simulink model "DABTestHarnessPlant"  (R2026a)
settings: Solver=ode23t  StopTime=5e-3  MaxStep=1e-5  AbsTol=1e-3
PreLoadFcn:
  | DABDefaultInputParameters;
model workspace (MAT data in the model file):
  ConverterKey = "DAB"
undefined symbols (not defined in the file or in its folder): DABController, DABDesign, DiscIntNeverNeededParam
libraries: ee_lib x45, nesl_utility x38, fl_lib x19, simulink_extras x1
(part 1 of 4)
settings Model: Creator=vsolaise  LastModifiedBy=vsolaise
settings SimscapeCC: SimscapeNominalValues="[{\"value\":\"1\",\"unit\":\"A\"},{\"value\":\"1\",\"unit\":\"bar\"},{\"value\":\"1\",\"unit\":\"cm^2\"},{\"value\":\"1\",\"unit\":\"cm^3/s\"},{\"value\":\"1\",\"unit\":\"kJ/kg\"},{\"value\":\"1\",\"unit\":\"kW\"},{\"value\":\"1\",\"unit\":\"l\"},{\"value\":\"1\",\"unit\":\"N\"},{\"value\":\"1\",\"unit\":\"N*m\"},{\"value\":\"1\",\"unit\":\"V\"}]"  SimscapeLogName=simlogDABConverter  SimscapeLogDataHistory=5000.0

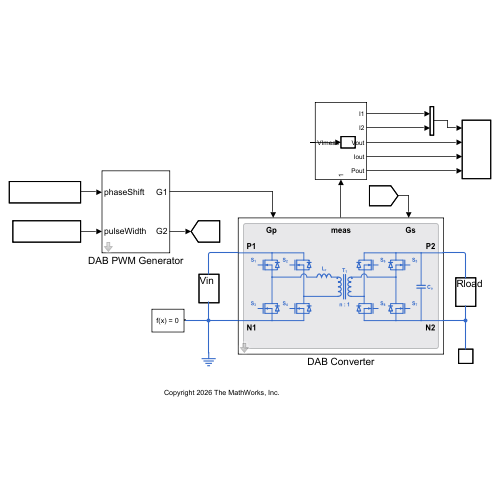
[thumbnail: Simulink's stored preview of the top-level diagram]
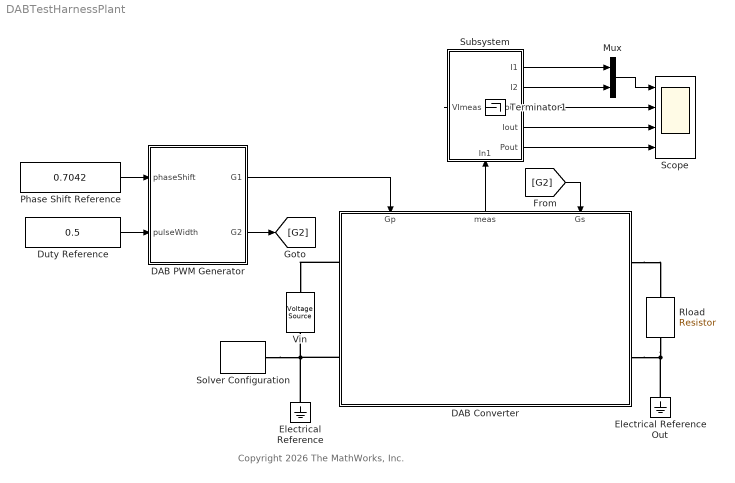
== system DABTestHarnessPlant ==
  note: Copyright 2026 The MathWorks, Inc.
  DAB Converter : Subsystem  mask(Dual Active Bridge DC-DC Converter){modelOption=Simplified, ratedPower=10000, ratedPower_unit=W, Vin=750, Vin_unit=V, Vout=525, Vout_unit=V, Fsw=100000, Fsw_unit=Hz, turnsRatio=1.4286, Co=2.963e-5, Co_unit=F, Rco=0.001, Rco_unit=mOhm, seriesInductorOption=Use transformer leakage inductance, Lr=0, Lr_unit=H, RLr=0.01, RLr_unit=Ohm, Lm=1.4062e-3, Lm_unit=H, Llk1=3.913e-5, Llk1_unit=H, RLlk1=0.01, RLlk1_unit=Ohm, Llk2=4.7935e-6, Llk2_unit=H, RLlk2=0.01, RLlk2_unit=Ohm, Vco=525, Vco_unit=V, switchDeviceOptionPri=MOSFET (Ideal, Switching) with Thermal, RdsOnPri=0.005, RdsOnPri_unit=Ohm, GdsOffPri=1e-5, GdsOffPri_unit=1/Ohm, VthPri=3, VthPri_unit=V, CossPri=2e-10, CossPri_unit=F, simTempPri=25, simTempPri_unit=degC, VfPri=0.005, VfPri_unit=V, RdPri=1, RdPri_unit=mOhm, GdPri=1e-5, GdPri_unit=1/Ohm, switchDeviceOptionSec=MOSFET (Ideal, Switching) with Thermal, RdsOnSec=0.005, RdsOnSec_unit=Ohm, GdsOffSec=1e-5, GdsOffSec_unit=1/Ohm, VthSec=3, VthSec_unit=V, CossSec=2e-10, CossSec_unit=F, simTempSec=25, simTempSec_unit=degC, VfSec=0.005, VfSec_unit=V, RdSec=1, RdSec_unit=mOhm, GdSec=1e-5, GdSec_unit=1/Ohm}
      mask prompts: modelOption "Model option"; ratedPower "Rated power"; Vin "Nominal input voltage"; Vout "Nominal output voltage"; Fsw "Switching frequency"; turnsRatio "Transformer turns ratio (Np/Ns)"; Co "Secondary output capacitance"; Rco "Secondary output capacitance ESR"; seriesInductorOption "Series inductance"; Lr "Series inductance (Lr)"; RLr "Series inductance resistance"; Lm "Magnetizing inductance (Lm)"; Llk1 "Primary leakage inductance (Llk1)"; RLlk1 "Primary winding resistance"; Llk2 "Secondary leakage inductance (Llk2)"; RLlk2 "Secondary winding resistance"; Vco "Initial output capacitor voltage"; switchDeviceOptionPri "Switch device"; RdsOnPri "On-state resistance (RdsOn)"; GdsOffPri "Off-state conductance (GdsOff)"; VthPri "Threshold voltage"; CossPri "Output capacitance (Coss)"; simTempPri "Simulation temperature"; VfPri "Diode forward voltage (Vf)"; RdPri "Diode on resistance (Rd)"; GdPri "Diode off conductance (Gd)"; switchDeviceOptionSec "Switch device"; RdsOnSec "On-state resistance (RdsOn)"; GdsOffSec "Off-state conductance (GdsOff)"; VthSec "Threshold voltage"; CossSec "Output capacitance (Coss)"; simTempSec "Simulation temperature"; VfSec "Diode forward voltage (Vf)"; RdSec "Diode on resistance (Rd)"; GdSec "Diode off conductance (Gd)"
      mask help: Dual Active Bridge (DAB) DC-DC Converter with variant options for HDL and Simulation models.
      mask init:
      | %% Unit conversion: convert displayed values to base SI units
      | convMap = containers.Map( ...
      |     {'W','kW','MW','V','kV','mV','F','mF','uF','nF','pF', ...
      |      'H','mH','uH','nH','Ohm','kOhm','mOhm','S','mS','1/Ohm', ...
      |      'Hz','kHz','MHz'}, ...
      |     {1, 1e3, 1e6, 1, 1e3, 1e-3, 1, 1e-3, 1e-6, 1e-9, 1e-12, ...
      |      1, 1e-3, 1e-6, 1e-9, 1, 1e3, 1e-3, 1, 1e-3, 1, ...
      |      1, 1e3, 1e6});
      | 
      | ratedPower_SI = ratedPower * convMap(ratedPower_unit);
      | Vin_SI = Vin * convMap(Vin_unit);
      | Vout_SI = Vout * convMap(Vout_unit);
      | Fsw_SI = Fsw * convMap(Fsw_unit);
      | Llk1_SI = Llk1 * convMap(Llk1_unit);
      | RLlk1_SI = RLlk1 * convMap(RLlk1_unit);
      | Llk2_SI = Llk2 * convMap(Llk2_unit);
      | RLlk2_SI = RLlk2 * convMap(RLlk2_unit);
      | Lr_SI = Lr * convMap(Lr_unit);
      | RLr_SI = RLr * convMap(RLr_unit);
      | % When the model compiles, the transformer leakages must be positive, and so must Lr when the
      | % external inductor is used. A dialog change is not checked, so Lr can be entered after the option.
      | if any(strcmp(get_param(bdroot(gcb), 'SimulationStatus'), {'updating', 'initializing'}))
      |     if ~(isfinite(Llk1_SI) && Llk1_SI > 0 && isfinite(Llk2_SI) && Llk2_SI > 0)
      |         error('The transformer leakage inductances must be positive. Primary: %g H, secondary: %g H.', Llk1_SI, Llk2_SI);
      |     end
      |     if strcmp(get_param(gcb, 'seriesInductorOption'), 'Use external inductance') && ~(isfinite(Lr_SI) && Lr_SI > 0)
      |         error('The external series inductance must be positive when it is used. Lr: %g H.', Lr_SI);
      |     end
      | end
      | Lm_SI = Lm * convMap(Lm_unit);
      | Co_SI = Co * convMap(Co_unit);
      | Rco_SI = Rco * convMap(Rco_unit);
      | Vco_SI = Vco * convMap(Vco_unit);
      | 
      | %% Primary switch params
      | RdsOnPri_SI = RdsOnPri * convMap(RdsOnPri_unit);
      | GdsOffPri_SI = GdsOffPri * convMap(GdsOffPri_unit);
      | VthPri_SI = VthPri * convMap(VthPri_unit);
      | CossPri_SI = CossPri * convMap(CossPri_unit);
      | 
      | %% Secondary switch params
      | RdsOnSec_SI = RdsOnSec * convMap(RdsOnSec_unit);
      | GdsOffSec_SI = GdsOffSec * convMap(GdsOffSec_unit);
      | VthSec_SI = VthSec * convMap(VthSec_unit);
      | CossSec_SI = CossSec * convMap(CossSec_unit);
      | 
      | %% Primary switch protection-diode params
      | VfPri_SI = VfPri * convMap(VfPri_unit);
      | RdPri_SI = RdPri * convMap(RdPri_unit);
      | GdPri_SI = GdPri * convMap(GdPri_unit);
      | 
      | %% Secondary switch protection-diode params
      | VfSec_SI = VfSec * convMap(VfSec_unit);
      | RdSec_SI = RdSec * convMap(RdSec_unit);
      | GdSec_SI = GdSec * convMap(GdSec_unit);
      | 
      | 
      | %% Simulation temperature (thermal MOSFET)
      | % Temperature is an OFFSET unit (K = degC + 273.15), so it cannot use the
      | % multiplicative convMap; convert it explicitly. These Kelvin variables are
      | % read directly by each thermal MOSFET device junction-temperature target and
      | % by each bridge Temperature Source.
      | if strcmp(simTempPri_unit, 'degC')
      |     simTempPri_K = simTempPri + 273.15;
      | else
      |     simTempPri_K = simTempPri;
      | end
      | if strcmp(simTempSec_unit, 'degC')
      |     simTempSec_K = simTempSec + 273.15;
      | else
      |     simTempSec_K = simTempSec;
      | end
      | 
      | %% Apply variant selection
      | selectDABConverterModelOption(gcb);
      settings: CopyFcn="set_param(gcbh,\"LinkStatus\",\"none\");"  PortSchema="{\"entries\":[{\"content\":{\"sides\":[{\"content\":{\"connectorIds\":[\"LConn1\",\"LConn2\"]},\"type\":\"ConnectorPlacement.EquallySpacedRectSide\",\"uuid\":\"5eb81d01-b33d-480d-b92b-9ee197a9667d\"},{\"content\":{\"connectorIds\":[\"RConn1\",\"RConn2\"],\"side\":\"RIGHT\"},\"type\":\"ConnectorPlacement.EquallySpacedRectSide\",\"uuid\":\"a719554b-e33a-474b-8c80-408706add5ae\"},{\"content\":{\"connectorIds\":[\"In1\",\"Out1\",\"In2\"],\"side\":\"TOP\"},\"type\":\"ConnectorPlacement.EquallySpacedRectSide\",\"uuid\":\"aea510b9-aefe-49d3-b91f-0f6ebd0a6b41\"}]},\"type\":\"ConnectorPlacement.EquallySpacedConnector\",\"uuid\":\"00bcdd44-1110-449b-876a-23d9733cbf45\"}],\"packageUris\":[\"http://schema.mathworks.com/mf0/Connector/R2020b\"],\"version\":\"1.0\"}"
      mask Help: web('DABConverter.html')
      mask TypeOptions modelOption: Simplified | Detailed
      mask Callback modelOption: selectDABConverterModelOption(gcb);
      mask TypeOptions ratedPower_unit: W | kW | MW
      mask TypeOptions Vin_unit: mV | V | kV
      mask TypeOptions Vout_unit: mV | V | kV
      mask TypeOptions Fsw_unit: Hz | kHz | MHz
      mask TypeOptions Co_unit: F | mF | uF | nF | pF
      mask TypeOptions Rco_unit: mOhm | Ohm | kOhm
      mask TypeOptions seriesInductorOption: Use external inductance | Use transformer leakage inductance
      mask Callback seriesInductorOption: selectDABSeriesInductor(gcb);
      mask TypeOptions Lr_unit: H | mH | uH | nH
      mask TypeOptions RLr_unit: mOhm | Ohm | kOhm
      mask TypeOptions Lm_unit: H | mH | uH | nH
      mask TypeOptions Llk1_unit: H | mH | uH | nH
      mask TypeOptions RLlk1_unit: mOhm | Ohm | kOhm
      mask TypeOptions Llk2_unit: H | mH | uH | nH
      mask TypeOptions RLlk2_unit: mOhm | Ohm | kOhm
      mask TypeOptions Vco_unit: V | kV | mV
      mask TypeOptions switchDeviceOptionPri: Ideal Switch | MOSFET (Ideal, Switching) with Thermal
      mask Callback switchDeviceOptionPri: selectDABConverterSwitchDevice(gcb)
      mask TypeOptions RdsOnPri_unit: mOhm | Ohm | kOhm
      mask TypeOptions GdsOffPri_unit: S | mS | 1/Ohm
      mask TypeOptions VthPri_unit: mV | V | kV
      mask TypeOptions CossPri_unit: F | mF | uF | nF | pF
      mask TypeOptions simTempPri_unit: degC | K
      mask TypeOptions VfPri_unit: mV | V | kV
      mask TypeOptions RdPri_unit: mOhm | Ohm | kOhm
      mask TypeOptions GdPri_unit: S | mS | 1/Ohm
      mask TypeOptions switchDeviceOptionSec: Ideal Switch | MOSFET (Ideal, Switching) with Thermal
      mask Callback switchDeviceOptionSec: selectDABConverterSwitchDevice(gcb)
      mask TypeOptions RdsOnSec_unit: mOhm | Ohm | kOhm
      mask TypeOptions GdsOffSec_unit: S | mS | 1/Ohm
      mask TypeOptions VthSec_unit: mV | V | kV
      mask TypeOptions CossSec_unit: F | mF | uF | nF | pF
      mask TypeOptions simTempSec_unit: degC | K
      mask TypeOptions VfSec_unit: mV | V | kV
      mask TypeOptions RdSec_unit: mOhm | Ohm | kOhm
      mask TypeOptions GdSec_unit: S | mS | 1/Ohm
      mask DialogControl DABConverterParameters Prompt: DAB Converter Parameters
      mask DialogControl TransformerParameters Prompt: Transformer
      mask DialogControl PrimarySwitch Prompt: Primary Switch
      mask DialogControl openMOSFETPriMask Prompt: Open MOSFET block mask
      mask DialogControl openMOSFETPriMask Callback: open_system([gcb '/DABConverterVariant/DetailedModel/PrimaryBridge/SwitchingMOSFETwithThermal/MOSFETPriA1'], 'mask')
      mask DialogControl applyMOSFETPriParam Prompt: Apply parameters to all primary MOSFET blocks
      mask DialogControl applyMOSFETPriParam Callback: applyDABConverterMOSFETParameters(gcb, 'primary')
      mask DialogControl SecondarySwitch Prompt: Secondary Switch
      mask DialogControl openMOSFETSecMask Prompt: Open MOSFET block mask
      mask DialogControl openMOSFETSecMask Callback: open_system([gcb '/DABConverterVariant/DetailedModel/SecondaryBridge/SwitchingMOSFETwithThermal/MOSFETSecA1'], 'mask')
      mask DialogControl applyMOSFETSecParam Prompt: Apply parameters to all secondary MOSFET blocks
      mask DialogControl applyMOSFETSecParam Callback: applyDABConverterMOSFETParameters(gcb, 'secondary')
      mask DialogControl ExportPanel Prompt: Export to Unmasked Subsystem
      mask DialogControl ExportInfo Prompt: To customize the converter, export it as an unmasked subsystem with the active variant flattened - a standalone, fully-editable circuit plus a parameter file. Requires the "Variant Manager for Simulink" add-on.
      mask DialogControl exportToModel Prompt: Export
      mask DialogControl exportToModel Callback: exportConverterModelFromMask(gcb);
      mask Display: image('DABConverterIcon.svg');
  DAB PWM Generator : Subsystem  mask(Dual Active Bridge PWM Generator){solverMode=Variable-step (continuous), Ts=1e-8, Fsw=DABDesign.switchingFrequency.value, Tdead=DABDesign.deadTime.value, primaryGateVoltageOn=DABController.gateVoltage, primaryGateVoltageOff=0, secondaryGateVoltageOn=DABController.gateVoltage, secondaryGateVoltageOff=0}
      mask prompts: solverMode "Solver mode"; Ts "Sample time (s)"; Fsw "Switching frequency (Hz)"; Tdead "Dead time (s)"; primaryGateVoltageOn "Primary bridge gate ON voltage (V)"; primaryGateVoltageOff "Primary bridge gate OFF voltage (V)"; secondaryGateVoltageOn "Secondary bridge gate ON voltage (V)"; secondaryGateVoltageOff "Secondary bridge gate OFF voltage (V)"
      mask help:
      | This block generates dual-active-bridge PWM gate signals with a dead time from a commanded phase shift.
      |
      | For a variable-step solver, set Solver mode to Variable-step (continuous). For a fixed-step solver, set Solver mode to Fixed-step (discrete) and set Sample time to a positive value.
      mask init:
      | % Solver mode. Switch every sawtooth ramp in this block between its continuous
      | % and its discrete implementation, and show the sample time only when it is used.
      | pwmGeneratorBlock = gcb;
      | if strcmp(get_param(pwmGeneratorBlock, 'solverMode'), 'Fixed-step (discrete)')
      |     pwmGeneratorRampChoice = 'FixedStep';
      |     pwmGeneratorSampleTimeVisibility = 'on';
      | else
      |     pwmGeneratorRampChoice = 'VariableStep';
      |     pwmGeneratorSampleTimeVisibility = 'off';
      | end
      | 
      | % A block may hold more than one ramp, at any depth, so the ramps are found by the
      | % "Ramp Mode" suffix on their names rather than by one fixed path. The match filter
      | % keeps every variant choice in the search, which is also what silences the
      | % find_system default-variants warning.
      | pwmGeneratorRamps = find_system(pwmGeneratorBlock, ...
      |     'MatchFilter', @Simulink.match.allVariants, 'LookUnderMasks', 'all', ...
      |     'FollowLinks', 'on', 'Regexp', 'on', 'BlockType', 'SubSystem', ...
      |     'Name', 'Ramp Mode$');
      | for pwmGeneratorRampIndex = 1:numel(pwmGeneratorRamps)
      |     set_param(pwmGeneratorRamps{pwmGeneratorRampIndex}, ...
      |         'LabelModeActiveChoice', pwmGeneratorRampChoice);
      | end
      | 
      | % Only the discrete ramp declares a rate, so the sample time is hidden in the
      | % continuous mode. The guard keeps the code silent on a mask still being built.
      | pwmGeneratorMask = Simulink.Mask.get(pwmGeneratorBlock);
      | pwmGeneratorSampleTime = pwmGeneratorMask.getParameter('Ts');
      | if ~isempty(pwmGeneratorSampleTime)
      |     pwmGeneratorSampleTime.Visible = pwmGeneratorSampleTimeVisibility;
      | end
      mask Help: web('DABPWMGenerator.html')
      mask TypeOptions solverMode: Variable-step (continuous) | Fixed-step (discrete)
      mask Callback solverMode:
      | % Solver mode. Switch every sawtooth ramp in this block between its continuous
      | % and its discrete implementation, and show the sample time only when it is used.
      | pwmGeneratorBlock = gcb;
      | if strcmp(get_param(pwmGeneratorBlock, 'solverMode'), 'Fixed-step (discrete)')
      |     pwmGeneratorRampChoice = 'FixedStep';
      |     pwmGeneratorSampleTimeVisibility = 'on';
      | else
      |     pwmGeneratorRampChoice = 'VariableStep';
      |     pwmGeneratorSampleTimeVisibility = 'off';
      | end
      | 
      | % A block may hold more than one ramp, at any depth, so the ramps are found by the
      | % "Ramp Mode" suffix on their names rather than by one fixed path. The match filter
      | % keeps every variant choice in the search, which is also what silences the
      | % find_system default-variants warning.
      | pwmGeneratorRamps = find_system(pwmGeneratorBlock, ...
      |     'MatchFilter', @Simulink.match.allVariants, 'LookUnderMasks', 'all', ...
      |     'FollowLinks', 'on', 'Regexp', 'on', 'BlockType', 'SubSystem', ...
      |     'Name', 'Ramp Mode$');
      | for pwmGeneratorRampIndex = 1:numel(pwmGeneratorRamps)
      |     set_param(pwmGeneratorRamps{pwmGeneratorRampIndex}, ...
      |         'LabelModeActiveChoice', pwmGeneratorRampChoice);
      | end
      | 
      | % Only the discrete ramp declares a rate, so the sample time is hidden in the
      | % continuous mode. The guard keeps the code silent on a mask still being built.
      | pwmGeneratorMask = Simulink.Mask.get(pwmGeneratorBlock);
      | pwmGeneratorSampleTime = pwmGeneratorMask.getParameter('Ts');
      | if ~isempty(pwmGeneratorSampleTime)
      |     pwmGeneratorSampleTime.Visible = pwmGeneratorSampleTimeVisibility;
      | end
      mask DialogControl DescTextVar Prompt:
      | This block generates dual-active-bridge PWM gate signals with a dead time from a commanded phase shift.
      | 
      | For a variable-step solver, set Solver mode to Variable-step (continuous). For a fixed-step solver, set Solver mode to Fixed-step (discrete) and set Sample time to a positive value.
      mask DialogControl SolverPanel Prompt: Solver Settings
      mask DialogControl SwitchingPanel Prompt: Switching Parameters
      mask DialogControl GateDrivePanel Prompt: Gate Drive
  Duty Reference : Constant  Value=0.5
  Electrical Reference : fl_lib/Electrical/Electrical Elements/Electrical Reference
  Electrical Reference Out : fl_lib/Electrical/Electrical Elements/Electrical Reference
  Mux : Mux  Inputs=2
  Phase Shift Reference : Constant  Value=0.7042
  Rload : fl_lib/Electrical/Electrical Elements/Resistor  R=27.5625 Ohm  i_specify=off  i_priority=None  i=0 A  i_nominal_specify=off  i_nominal_value=1  i_nominal_unit=A  v_specify=off  v_priority=None  v=0 V  v_nominal_specify=off  v_nominal_value=1  v_nominal_unit=V
  Scope : Scope  NumInputPorts=4
      settings: Title=Output Voltage (V)  ActiveDisplayYMinimum=384.33567337339571  ActiveDisplayYMaximum=543.59763143317582
  Solver Configuration : nesl_utility/Solver Configuration  PhysicalDomain=network_engine_domain  SubClassName=solver  LeftPortType=input  RightPortType=generic  Tones=[]  Harmonics=[]  SimulateNoise=off  Profile=off  UseLocalSampling=off  EnableSwitchedLinearOptims=on  FrequencyDomain=off  UseCCode=off  RelTol=0.001  AbsTol=0.001  MinStep=1e-09  ToWorkspace=off  RevertToSquareIcSolve=off  NumHomotopyIterations=100  PhasorMode=off  PhasorModeNumHarmonics=1  ConsistencySolver=NEWTON_XTOL_AFTER_FTOL  CanonicalOrdering=UNORDERED  OptimizeIntermediates=UNOPTIMIZED  IndexReductionMethod=DerivativeReplacement  DoDC=off  ResidualTolerance=1e-09  ConsistencyTolSource=GLOBAL  ConsistencyAbsTol=0.001  ConsistencyRelTol=0.001  ConsistencyTolFactor=0.001  UseLocalSolver=on  LocalSolverChoice=NE_BACKWARD_EULER_ADVANCER  ResolveIndetEquations=on  FunctionEvalNumThread=1  LocalSolverSampleTime=1e-7  DoFixedCost=on  MaxNonlinIter=6  MaxModeIter=2  ComputeImpulses=off  ImpulseIterations=2  LinearAlgebra=auto  LinearAlgebraNumThread=0  EquationFormulation=NE_TIME_EF  DelaysMemoryBudget=1024  AutomaticFiltering=on  FilteringTimeConstant=0.001  PartitionStorageMethod=AS_NEEDED  PartitionMemoryBudget=1024  PartitionMethod=ROBUST  MultibodyUseLocalSolver=off  MultibodyLocalSolverChoice=ODE1  MultibodyLocalSolverSampleTime=0.001
  Subsystem : Subsystem
      settings: PortSchema="{\"entries\":[{\"content\":{\"sides\":[{\"content\":{\"connectorIds\":[\"Out6\"]},\"type\":\"ConnectorPlacement.EquallySpacedRectSide\",\"uuid\":\"f2b899f7-a6f0-4063-b280-75fc43e532d5\"},{\"content\":{\"connectorIds\":[\"Out1\",\"Out2\",\"Out3\",\"Out4\",\"Out5\"],\"side\":\"RIGHT\"},\"type\":\"ConnectorPlacement.EquallySpacedRectSide\",\"uuid\":\"5de70531-a79e-4c62-9cd6-16ab34a78e6e\"},{\"content\":{\"side\":\"TOP\"},\"type\":\"ConnectorPlacement.EquallySpacedRectSide\",\"uuid\":\"e5bc4a57-59c4-404a-a3d7-aeb4f7590bd8\"},{\"content\":{\"connectorIds\":[\"In1\"],\"side\":\"BOTTOM\"},\"type\":\"ConnectorPlacement.EquallySpacedRectSide\",\"uuid\":\"d1dcebc2-7af2-4d54-9158-2e062e509fbc\"}]},\"type\":\"ConnectorPlacement.EquallySpacedConnector\",\"uuid\":\"ad567749-1bde-47d1-aaf1-1f8d8a2cad80\"}],\"packageUris\":[\"http://schema.mathworks.com/mf0/Connector/R2020b\"],\"version\":\"1.0\"}"
  Terminator1 : Terminator
  Vin : ee_lib/Sources/Voltage Source  dc_voltage=750 V  ac_voltage=0 V  ac_shift=0 rad  ac_frequency=60 Hz  noise_mode=ee.enum.sources.noise.Disabled  PSD=0 V^2/Hz  sample_time=1e-3 s  repeatability=ee.enum.sources.repeatability.NotRepeatable  user_seed=0  auto_seed=1556750757  i_specify=off  i_priority=None  i=0 A  i_nominal_specify=off  i_nominal_value=1  i_nominal_unit=A  v_specify=off  v_priority=None  v=0 V  v_nominal_specify=off  v_nominal_value=1  v_nominal_unit=V
  wires:
  Subsystem/1(I1) -> Mux/1
  Subsystem/2(I2) -> Mux/2
  DAB Converter/1(meas) -> Subsystem/1(In1)
  Subsystem/3(Vout) -> Scope/2
  Mux/1 -> Scope/1
  Subsystem/4(Iout) -> Scope/3
  Subsystem/5(Pout) -> Scope/4
  Phase Shift Reference/1 -> DAB PWM Generator/1(phaseShift)
  Duty Reference/1 -> DAB PWM Generator/2(pulseWidth)
  DAB PWM Generator/1(G1) -> DAB Converter/1(Gp)
  Subsystem/6(VImeas) -> Terminator1/1
  DAB PWM Generator/2(G2) -> [G2]
  [G2] -> DAB Converter/2(Gs)
  connections:
  DAB Converter/LConn1 -- Vin/LConn1
  DAB Converter/RConn1 -- Rload/LConn1
  Solver Configuration/RConn1 -- Electrical Reference/LConn1 -- DAB Converter/LConn2 -- Vin/RConn1
  Rload/RConn1 -- Electrical Reference Out/LConn1 -- DAB Converter/RConn2

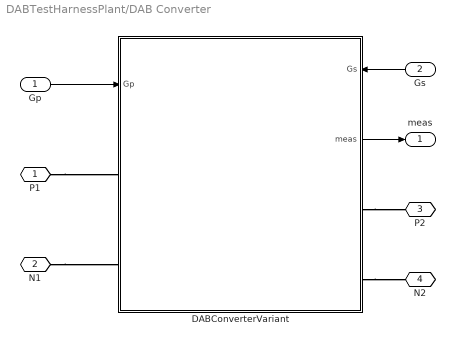
== system DABTestHarnessPlant/DAB Converter ==
  Gp : Inport
  Gs : Inport  Port=2
  DABConverterVariant : Subsystem  Variant=on  VariantControlMode=label  LabelModeActiveChoice=SimplifiedModel
      settings: PortSchema="{\"entries\":[{\"content\":{\"sides\":[{\"content\":{\"connectorIds\":[\"In1\",\"LConn1\",\"LConn2\"]},\"type\":\"ConnectorPlacement.EquallySpacedRectSide\",\"uuid\":\"6f245ee7-ecea-433e-8ace-55b7238b8bbd\"},{\"content\":{\"connectorIds\":[\"In2\",\"Out1\",\"RConn1\",\"RConn2\"],\"side\":\"RIGHT\"},\"type\":\"ConnectorPlacement.EquallySpacedRectSide\",\"uuid\":\"af7f8c88-8cd1-4285-8228-b98ea57f06ae\"},{\"content\":{\"side\":\"TOP\"},\"type\":\"ConnectorPlacement.EquallySpacedRectSide\",\"uuid\":\"820d378e-11b2-4797-9989-1ab18f65f7f5\"}]},\"type\":\"ConnectorPlacement.EquallySpacedConnector\",\"uuid\":\"ae0f71da-cdc3-4120-89e7-21ff59b441bf\"}],\"packageUris\":[\"http://schema.mathworks.com/mf0/Connector/R2020b\"],\"version\":\"1.0\"}"
  P1 : PMIOPort  Side=Left
  N1 : PMIOPort  Port=2  Side=Left
  P2 : PMIOPort  Port=3  Side=Right
  N2 : PMIOPort  Port=4  Side=Right
  meas : Outport
  wires:
  Gp/1 -> DABConverterVariant/1(Gp)
  Gs/1 -> DABConverterVariant/2(Gs)
  DABConverterVariant/1(meas) -> meas/1
  connections:
  DABConverterVariant/RConn2 -- N2/RConn1
  DABConverterVariant/RConn1 -- P2/RConn1
  N1/RConn1 -- DABConverterVariant/LConn2
  P1/RConn1 -- DABConverterVariant/LConn1

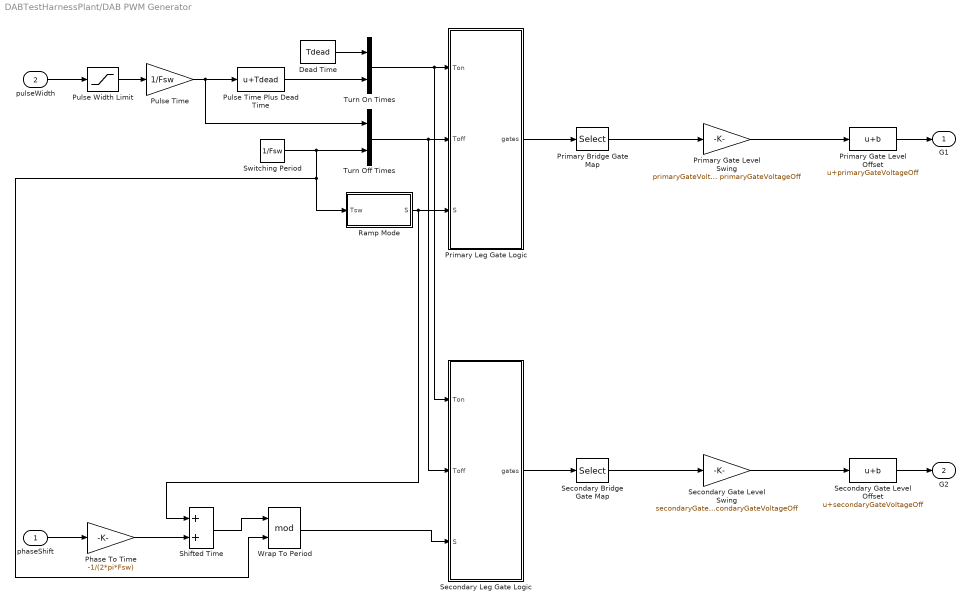
== system DABTestHarnessPlant/DAB PWM Generator ==
  phaseShift : Inport
  pulseWidth : Inport  Port=2
  Dead Time : Constant  Value=Tdead
  Phase To Time : Gain  Gain=-1/(2*pi*Fsw)
  Primary Bridge Gate Map : Selector  InputPortWidth=2  IndexOptions=Index vector (dialog)  Indices=[1 2 2 1]  OutputSizes=1
  Primary Gate Level Offset : Bias  Bias=primaryGateVoltageOff
  Primary Gate Level Swing : Gain  Gain=primaryGateVoltageOn - primaryGateVoltageOff
  Primary Leg Gate Logic : Subsystem
  Pulse Time : Gain  Gain=1/Fsw
  Pulse Time Plus Dead Time : Bias  Bias=Tdead
  Pulse Width Limit : Saturate  UpperLimit=1 - Tdead*Fsw  LowerLimit=Tdead*Fsw
  Ramp Mode : Subsystem  Variant=on  VariantControlMode=label  LabelModeActiveChoice=VariableStep
  Secondary Bridge Gate Map : Selector  InputPortWidth=2  IndexOptions=Index vector (dialog)  Indices=[1 2 2 1]  OutputSizes=1
  Secondary Gate Level Offset : Bias  Bias=secondaryGateVoltageOff
  Secondary Gate Level Swing : Gain  Gain=secondaryGateVoltageOn - secondaryGateVoltageOff
  Secondary Leg Gate Logic : Subsystem
  Shifted Time : Sum
  Switching Period : Constant  Value=1/Fsw
  Turn Off Times : Mux  Inputs=2
  Turn On Times : Mux  Inputs=2
  Wrap To Period : Math  Operator=mod
  G1 : Outport
  G2 : Outport  Port=2
  wires:
  Secondary Gate Level Offset/1 -> G2/1
  Primary Gate Level Offset/1 -> G1/1
  Secondary Bridge Gate Map/1 -> Secondary Gate Level Swing/1
  Secondary Leg Gate Logic/1(gates) -> Secondary Bridge Gate Map/1
  Primary Bridge Gate Map/1 -> Primary Gate Level Swing/1
  Primary Leg Gate Logic/1(gates) -> Primary Bridge Gate Map/1
  Wrap To Period/1 -> Secondary Leg Gate Logic/3(S)
  Shifted Time/1 -> Wrap To Period/1
  Phase To Time/1 -> Shifted Time/2
  phaseShift/1 -> Phase To Time/1
  Ramp Mode/1(S) -> Shifted Time/1, Primary Leg Gate Logic/3(S)
  Turn Off Times/1 -> Secondary Leg Gate Logic/2(Toff), Primary Leg Gate Logic/2(Toff)
  Turn On Times/1 -> Secondary Leg Gate Logic/1(Ton), Primary Leg Gate Logic/1(Ton)
  Secondary Gate Level Swing/1 -> Secondary Gate Level Offset/1
  Primary Gate Level Swing/1 -> Primary Gate Level Offset/1
  Switching Period/1 -> Wrap To Period/2, Ramp Mode/1(Tsw), Turn Off Times/2
  Pulse Time Plus Dead Time/1 -> Turn On Times/2
  Dead Time/1 -> Turn On Times/1
  Pulse Time/1 -> Turn Off Times/1, Pulse Time Plus Dead Time/1
  Pulse Width Limit/1 -> Pulse Time/1
  pulseWidth/1 -> Pulse Width Limit/1

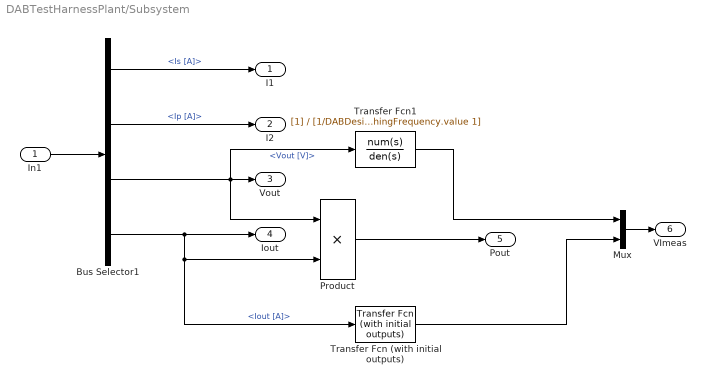
== system DABTestHarnessPlant/Subsystem ==
  In1 : Inport
  Bus Selector1 : BusSelector  OutputSignals=Is [A],Ip [A],Vout [V],Iout [A]
  Mux : Mux  Inputs=2
  Product : Product
  Transfer Fcn (with initial outputs) : simulink_extras/Additional Linear/Transfer Fcn (with initial outputs)  N=[1]  D=[1/DABDesign.switchingFrequency.value 1]  Y0=DABDesign.V2nom.value  U0=DABDesign.V2nom.value
  Transfer Fcn1 : TransferFcn  Denominator=[1/DABDesign.switchingFrequency.value 1]
  I1 : Outport
  I2 : Outport  Port=2
  Vout : Outport  Port=3
  Iout : Outport  Port=4
  Pout : Outport  Port=5
  VImeas : Outport  Port=6
  wires:
  In1/1 -> Bus Selector1/1
  Bus Selector1/1 -> I1/1  "<Is [A]>"
  Bus Selector1/2 -> I2/1  "<Ip [A]>"
  Product/1 -> Pout/1
  Bus Selector1/3 -> Transfer Fcn1/1, Vout/1, Product/1  "<Vout [V]>"
  Bus Selector1/4 -> Transfer Fcn (with initial outputs)/1, Product/2, Iout/1  "<Iout [A]>"
  Transfer Fcn (with initial outputs)/1 -> Mux/2
  Transfer Fcn1/1 -> Mux/1
  Mux/1 -> VImeas/1

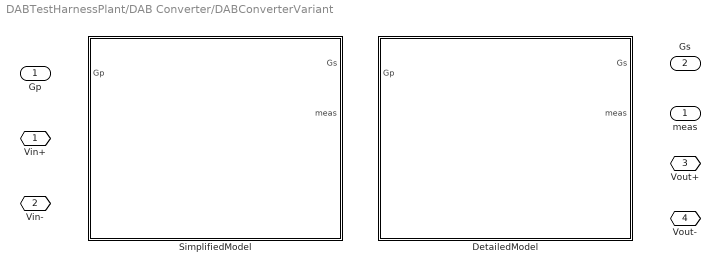
== system DABTestHarnessPlant/DAB Converter/DABConverterVariant ==
  Gp : Inport
  Gs : Inport  Port=2
  DetailedModel : Subsystem  VariantControl=DetailedModel
      settings: PortSchema="{\"entries\":[{\"content\":{\"sides\":[{\"content\":{\"connectorIds\":[\"In1\",\"LConn1\",\"LConn2\"]},\"type\":\"ConnectorPlacement.EquallySpacedRectSide\",\"uuid\":\"6f245ee7-ecea-433e-8ace-55b7238b8bbd\"},{\"content\":{\"connectorIds\":[\"In2\",\"Out1\",\"RConn1\",\"RConn2\"],\"side\":\"RIGHT\"},\"type\":\"ConnectorPlacement.EquallySpacedRectSide\",\"uuid\":\"af7f8c88-8cd1-4285-8228-b98ea57f06ae\"},{\"content\":{\"side\":\"TOP\"},\"type\":\"ConnectorPlacement.EquallySpacedRectSide\",\"uuid\":\"820d378e-11b2-4797-9989-1ab18f65f7f5\"}]},\"type\":\"ConnectorPlacement.EquallySpacedConnector\",\"uuid\":\"ae0f71da-cdc3-4120-89e7-21ff59b441bf\"}],\"packageUris\":[\"http://schema.mathworks.com/mf0/Connector/R2020b\"],\"version\":\"1.0\"}"
  SimplifiedModel : Subsystem  VariantControl=SimplifiedModel
      settings: PortSchema="{\"entries\":[{\"content\":{\"sides\":[{\"content\":{\"connectorIds\":[\"In1\",\"LConn1\",\"LConn2\"]},\"type\":\"ConnectorPlacement.EquallySpacedRectSide\",\"uuid\":\"6f245ee7-ecea-433e-8ace-55b7238b8bbd\"},{\"content\":{\"connectorIds\":[\"In2\",\"Out1\",\"RConn1\",\"RConn2\"],\"side\":\"RIGHT\"},\"type\":\"ConnectorPlacement.EquallySpacedRectSide\",\"uuid\":\"af7f8c88-8cd1-4285-8228-b98ea57f06ae\"},{\"content\":{\"side\":\"TOP\"},\"type\":\"ConnectorPlacement.EquallySpacedRectSide\",\"uuid\":\"820d378e-11b2-4797-9989-1ab18f65f7f5\"}]},\"type\":\"ConnectorPlacement.EquallySpacedConnector\",\"uuid\":\"ae0f71da-cdc3-4120-89e7-21ff59b441bf\"}],\"packageUris\":[\"http://schema.mathworks.com/mf0/Connector/R2020b\"],\"version\":\"1.0\"}"
  Vin+ : PMIOPort  Side=Left
  Vin- : PMIOPort  Port=2  Side=Left
  Vout+ : PMIOPort  Port=3  Side=Right
  Vout- : PMIOPort  Port=4  Side=Right
  meas : Outport

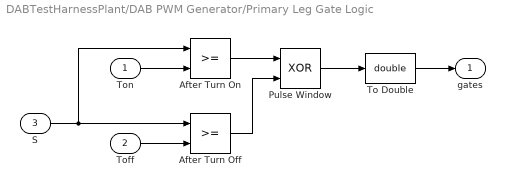
== system DABTestHarnessPlant/DAB PWM Generator/Primary Leg Gate Logic ==
  Ton : Inport
  Toff : Inport  Port=2
  S : Inport  Port=3
  After Turn Off : RelationalOperator
  After Turn On : RelationalOperator
  Pulse Window : Logic  Operator=XOR
  To Double : DataTypeConversion  OutDataTypeStr=double
  gates : Outport
  wires:
  To Double/1 -> gates/1
  Pulse Window/1 -> To Double/1
  After Turn Off/1 -> Pulse Window/2
  After Turn On/1 -> Pulse Window/1
  S/1 -> After Turn On/1, After Turn Off/1
  Toff/1 -> After Turn Off/2
  Ton/1 -> After Turn On/2

== system DABTestHarnessPlant/DAB PWM Generator/Ramp Mode ==
  Tsw : Inport
  FixedStep : Subsystem  VariantControl=FixedStep
  VariableStep : Subsystem  VariantControl=VariableStep
  S : Outport

== system DABTestHarnessPlant/DAB PWM Generator/Secondary Leg Gate Logic ==
  Ton : Inport
  Toff : Inport  Port=2
  S : Inport  Port=3
  After Turn Off : RelationalOperator
  After Turn On : RelationalOperator
  Pulse Window : Logic  Operator=XOR
  To Double : DataTypeConversion  OutDataTypeStr=double
  gates : Outport
  wires:
  To Double/1 -> gates/1
  Pulse Window/1 -> To Double/1
  After Turn Off/1 -> Pulse Window/2
  After Turn On/1 -> Pulse Window/1
  S/1 -> After Turn On/1, After Turn Off/1
  Toff/1 -> After Turn Off/2
  Ton/1 -> After Turn On/2

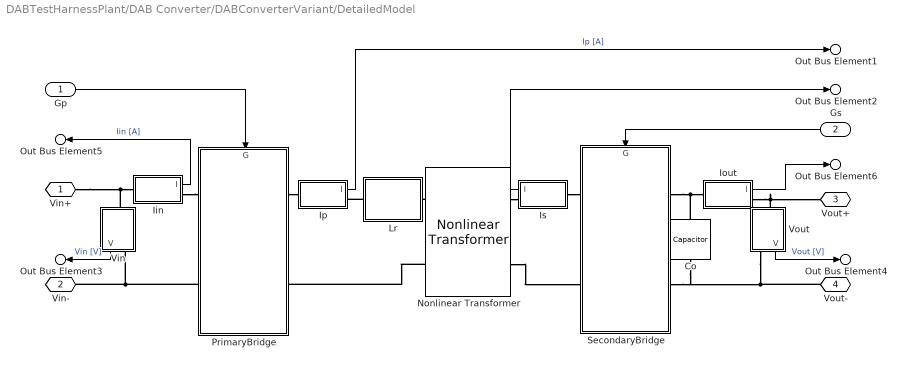
== system DABTestHarnessPlant/DAB Converter/DABConverterVariant/DetailedModel ==
  Gp : Inport
  Gs : Inport  Port=2
  Co : ee_lib/Passive/Capacitor  cap_option=ee.enum.passive.capacitor.capOption.const  c=Co_SI F  Cvec=[1e-05, 1e-06] F  Vvec=[0, 10] V  CV_table_symmetry=ee.enum.passive.capacitor.tableSymmetry.yes  f_vec=[1, 10] kHz  DFext_vec=[.8, 1.2]  enable_C_tol=ee.enum.toleranceApplication.none  averaging_period=0 s  C_tol=5  tol_distribution=ee.enum.toleranceDistribution.uniform  nSigma=4  r=Rco_SI Ohm  g=0 1/Ohm  enable_operating_limits=ee.enum.enable.no  operating_limit_action=ee.enum.passive.reportOpLim.warn  max_working_voltage_range=[-25, 25] V  power_rating=1 W  maxTemperature=85 degC  thermalEnable=false  thermalMass=1 J/K  i_specify=off  i_priority=None  i=0 A  i_nominal_specify=off  i_nominal_value=1  i_nominal_unit=A  v_specify=off  v_priority=None  v=0 V  v_nominal_specify=off  v_nominal_value=1  v_nominal_unit=V  vc_specify=on  vc_priority=High  vc=Vco_SI V  vc_nominal_specify=off  vc_nominal_value=1  vc_nominal_unit=V  T_specify=off  T_priority=None  T=298.15 K  T_nominal_specify=off  T_nominal_value=1  T_nominal_unit=K
  Iin : Subsystem
      mask Display: disp('I')
  Iout : Subsystem
      mask Display: disp('I')
  Ip : Subsystem
      mask Display: disp('I')
  Is : Subsystem
      settings: PortSchema="{\"entries\":[{\"content\":{\"sides\":[{\"content\":{\"connectorIds\":[\"Out1\",\"LConn1\"]},\"type\":\"ConnectorPlacement.EquallySpacedRectSide\",\"uuid\":\"da66b42d-39ba-4e5d-9b19-dc680792542d\"},{\"content\":{\"connectorIds\":[\"RConn1\"],\"side\":\"RIGHT\"},\"type\":\"ConnectorPlacement.EquallySpacedRectSide\",\"uuid\":\"9a34d54a-b1f0-405a-82c9-4333c7864e33\"},{\"content\":{\"side\":\"TOP\"},\"type\":\"ConnectorPlacement.EquallySpacedRectSide\",\"uuid\":\"3d98f795-d173-4072-aa84-47617691d0d7\"}]},\"type\":\"ConnectorPlacement.EquallySpacedConnector\",\"uuid\":\"cc1a3107-18f6-4c4b-a82f-56637250e4a4\"}],\"packageUris\":[\"http://schema.mathworks.com/mf0/Connector/R2020b\"],\"version\":\"1.0\"}"
      mask Display: disp('I')
  Lr : Subsystem  Variant=on  VariantControlMode=label  LabelModeActiveChoice=LeakageInductance
  Nonlinear Transformer : ee_lib/Passive/Transformers/Nonlinear Transformer  Nw=turnsRatio  Nw2=1  winding_param_option=2  Req=0 Ohm  Leq=0 H  R_1=RLlk1_SI Ohm  L_1=Llk1_SI H  R_2=RLlk2_SI Ohm  L_2=Llk2_SI H  averaging_period=0 s  R_m=15000 Ohm  parameterization_option=1  H_data=[0, 200, 400, 600, 800, 1000] A/m  B_data=[0, .81, 1.25, 1.42, 1.48, 1.49] T  length_effective=0.2 m  area_effective=2e-4 m^2  L=Lm_SI H  L_sat=1e-2 H  current_data=[0, .4, .8, 1.2, 1.6, 2] A  magnetic_flux_data=[0, .161, .25, .284, .295, .299] .* 1e-3 Wb  magnetic_flux_sat=1.6e-04 Wb  dBdH0=0.005 T*m/A  B1=1.49 T  H1=1000 A/m  c=0.1  K=200 A/m  alpha=1e-4  interpolation_option=1  Leq_i0=0 A  L1_i0=0 A  L2_i0=0 A  x0_option=1  i_L0=0 A  phi0=0 Wb  B0=0 T  H0=0 A/m  Leq_g=1e-9 1/Ohm  L1_g=1e-9 1/Ohm  L2_g=1e-9 1/Ohm
  PrimaryBridge : Subsystem  Variant=on  VariantControlMode=label  LabelModeActiveChoice=SwitchingMOSFETwithThermal
      settings: PortSchema="{\"entries\":[{\"content\":{\"sides\":[{\"content\":{\"connectorIds\":[\"LConn1\",\"LConn2\"]},\"type\":\"ConnectorPlacement.EquallySpacedRectSide\",\"uuid\":\"d98ab02e-eaff-433c-abe3-9c8832e30ad4\"},{\"content\":{\"connectorIds\":[\"RConn1\",\"RConn2\"],\"side\":\"RIGHT\"},\"type\":\"ConnectorPlacement.EquallySpacedRectSide\",\"uuid\":\"c0772040-dd18-4215-ab8f-2785b86fdc85\"},{\"content\":{\"connectorIds\":[\"In1\"],\"side\":\"TOP\"},\"type\":\"ConnectorPlacement.EquallySpacedRectSide\",\"uuid\":\"58c66fea-5b87-40d4-9fd7-49b3eaec4a75\"}]},\"type\":\"ConnectorPlacement.EquallySpacedConnector\",\"uuid\":\"277158f2-ac55-4232-8e6b-6b9d1c92778d\"}],\"packageUris\":[\"http://schema.mathworks.com/mf0/Connector/R2020b\"],\"version\":\"1.0\"}"
  SecondaryBridge : Subsystem  Variant=on  VariantControlMode=label  LabelModeActiveChoice=SwitchingMOSFETwithThermal
      settings: PortSchema="{\"entries\":[{\"content\":{\"sides\":[{\"content\":{\"connectorIds\":[\"LConn1\",\"LConn2\"]},\"type\":\"ConnectorPlacement.EquallySpacedRectSide\",\"uuid\":\"d98ab02e-eaff-433c-abe3-9c8832e30ad4\"},{\"content\":{\"connectorIds\":[\"RConn1\",\"RConn2\"],\"side\":\"RIGHT\"},\"type\":\"ConnectorPlacement.EquallySpacedRectSide\",\"uuid\":\"c0772040-dd18-4215-ab8f-2785b86fdc85\"},{\"content\":{\"connectorIds\":[\"In1\"],\"side\":\"TOP\"},\"type\":\"ConnectorPlacement.EquallySpacedRectSide\",\"uuid\":\"58c66fea-5b87-40d4-9fd7-49b3eaec4a75\"}]},\"type\":\"ConnectorPlacement.EquallySpacedConnector\",\"uuid\":\"277158f2-ac55-4232-8e6b-6b9d1c92778d\"}],\"packageUris\":[\"http://schema.mathworks.com/mf0/Connector/R2020b\"],\"version\":\"1.0\"}"
  Vin : Subsystem
      mask Display: disp('V')
  Vout : Subsystem
      settings: PortSchema="{\"entries\":[{\"content\":{\"sides\":[{\"content\":{\"connectorIds\":[\"LConn1\"]},\"type\":\"ConnectorPlacement.EquallySpacedRectSide\",\"uuid\":\"da66b42d-39ba-4e5d-9b19-dc680792542d\"},{\"content\":{\"connectorIds\":[\"RConn1\",\"Out1\"],\"side\":\"RIGHT\"},\"type\":\"ConnectorPlacement.EquallySpacedRectSide\",\"uuid\":\"9a34d54a-b1f0-405a-82c9-4333c7864e33\"},{\"content\":{\"side\":\"TOP\"},\"type\":\"ConnectorPlacement.EquallySpacedRectSide\",\"uuid\":\"3d98f795-d173-4072-aa84-47617691d0d7\"}]},\"type\":\"ConnectorPlacement.EquallySpacedConnector\",\"uuid\":\"cc1a3107-18f6-4c4b-a82f-56637250e4a4\"}],\"packageUris\":[\"http://schema.mathworks.com/mf0/Connector/R2020b\"],\"version\":\"1.0\"}"
      mask Display: disp('V')
  Vin+ : PMIOPort  Side=Left
  Vin- : PMIOPort  Port=2  Side=Left
  Vout+ : PMIOPort  Port=3  Side=Right
  Vout- : PMIOPort  Port=4  Side=Right
  Out Bus Element1 : Outport  PortName=meas  Element=Ip [A]
  Out Bus Element2 : Outport  PortName=meas  Element=Is [A]
  Out Bus Element3 : Outport  PortName=meas  Element=Vin [V]
  Out Bus Element4 : Outport  PortName=meas  Element=Vout [V]
  Out Bus Element5 : Outport  PortName=meas  Element=Iin [A]
  Out Bus Element6 : Outport  PortName=meas  Element=Iout [A]
  wires:
  Ip/1(I) -> Out Bus Element1/1  "Ip [A]"
  Vin/1(V) -> Out Bus Element3/1  "Vin [V]"
  Iin/1(I) -> Out Bus Element5/1  "Iin [A]"
  Iout/1(I) -> Out Bus Element6/1
  Is/1(I) -> Out Bus Element2/1
  Vout/1(V) -> Out Bus Element4/1  "Vout [V]"
  Gs/1 -> SecondaryBridge/1(G)
  Gp/1 -> PrimaryBridge/1(G)
  connections:
  Nonlinear Transformer/RConn2 -- SecondaryBridge/RConn2
  Is/RConn1 -- SecondaryBridge/RConn1
  Iin/RConn1 -- PrimaryBridge/LConn1
  PrimaryBridge/RConn1 -- Ip/LConn1
  Lr/LConn1 -- Ip/RConn1
  Nonlinear Transformer/LConn1 -- Lr/RConn1
  Nonlinear Transformer/LConn2 -- PrimaryBridge/RConn2
  Nonlinear Transformer/RConn1 -- Is/LConn1
  Iout/RConn1 -- Vout/LConn1 -- Vout+/RConn1
  PrimaryBridge/LConn2 -- Vin-/RConn1 -- Vin/RConn1
  Vin/LConn1 -- Vin+/RConn1 -- Iin/LConn1
  Vout/RConn1 -- Co/RConn1 -- SecondaryBridge/LConn2 -- Vout-/RConn1
  Iout/LConn1 -- SecondaryBridge/LConn1 -- Co/LConn1

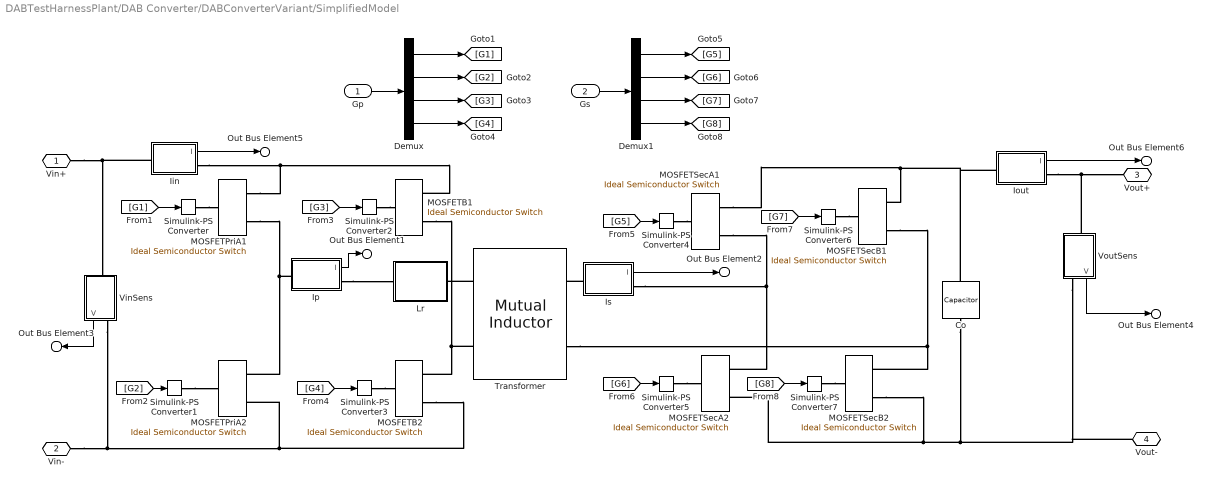
== system DABTestHarnessPlant/DAB Converter/DABConverterVariant/SimplifiedModel ==
  Gp : Inport
  Gs : Inport  Port=2
  Co : ee_lib/Passive/Capacitor  cap_option=ee.enum.passive.capacitor.capOption.const  c=Co_SI F  Cvec=[1e-05, 1e-06] F  Vvec=[0, 10] V  CV_table_symmetry=ee.enum.passive.capacitor.tableSymmetry.yes  f_vec=[1, 10] kHz  DFext_vec=[.8, 1.2]  enable_C_tol=ee.enum.toleranceApplication.none  averaging_period=0 s  C_tol=5  tol_distribution=ee.enum.toleranceDistribution.uniform  nSigma=4  r=Rco_SI Ohm  g=0 1/Ohm  enable_operating_limits=ee.enum.enable.no  operating_limit_action=ee.enum.passive.reportOpLim.warn  max_working_voltage_range=[-25, 25] V  power_rating=1 W  maxTemperature=85 degC  thermalEnable=false  thermalMass=1 J/K  i_specify=off  i_priority=None  i=0 A  i_nominal_specify=off  i_nominal_value=1  i_nominal_unit=A  v_specify=off  v_priority=None  v=0 V  v_nominal_specify=off  v_nominal_value=1  v_nominal_unit=V  vc_specify=on  vc_priority=High  vc=Vco_SI V  vc_nominal_specify=off  vc_nominal_value=1  vc_nominal_unit=V  T_specify=off  T_priority=None  T=298.15 K  T_nominal_specify=off  T_nominal_value=1  T_nominal_unit=K
  Demux : Demux
  Demux1 : Demux
  Iin : Subsystem
      mask Display: disp('I')
  Iout : Subsystem
      mask Display: disp('I')
  Ip : Subsystem
      mask Display: disp('I')
  Is : Subsystem
      mask Display: disp('I')
  Lr : Subsystem  Variant=on  VariantControlMode=label  LabelModeActiveChoice=LeakageInductance
  MOSFETB1 : ee_lib/Semiconductors & Converters/Ideal Semiconductor Switch  port_option=ee.enum.controlport.ps  Ron=RdsOnPri_SI Ohm  Goff=GdsOffPri_SI 1/Ohm  Vth=VthPri_SI V  diode_param=ee.enum.semiconductors.protectionDiode.nodynamics  diode_Vf=VfPri_SI V  diode_Ron=RdPri_SI Ohm  diode_Goff=GdPri_SI 1/Ohm  diode_C=50e-9 F  diode_iRM=-235 A  diode_iF=300 A  diode_idot=-50 A/us  diode_trr_param=ee.enum.converters.diodetrr.trr_factor  diode_trr_factor=3  diode_trr=15 us  diode_Qrr=1500 s*uA
  MOSFETB2 : ee_lib/Semiconductors & Converters/Ideal Semiconductor Switch  port_option=ee.enum.controlport.ps  Ron=RdsOnPri_SI Ohm  Goff=GdsOffPri_SI 1/Ohm  Vth=VthPri_SI V  diode_param=ee.enum.semiconductors.protectionDiode.nodynamics  diode_Vf=VfPri_SI V  diode_Ron=RdPri_SI Ohm  diode_Goff=GdPri_SI 1/Ohm  diode_C=50e-9 F  diode_iRM=-235 A  diode_iF=300 A  diode_idot=-50 A/us  diode_trr_param=ee.enum.converters.diodetrr.trr_factor  diode_trr_factor=3  diode_trr=15 us  diode_Qrr=1500 s*uA
  MOSFETPriA1 : ee_lib/Semiconductors & Converters/Ideal Semiconductor Switch  port_option=ee.enum.controlport.ps  Ron=RdsOnPri_SI Ohm  Goff=GdsOffPri_SI 1/Ohm  Vth=VthPri_SI V  diode_param=ee.enum.semiconductors.protectionDiode.nodynamics  diode_Vf=VfPri_SI V  diode_Ron=RdPri_SI Ohm  diode_Goff=GdPri_SI 1/Ohm  diode_C=50e-9 F  diode_iRM=-235 A  diode_iF=300 A  diode_idot=-50 A/us  diode_trr_param=ee.enum.converters.diodetrr.trr_factor  diode_trr_factor=3  diode_trr=15 us  diode_Qrr=1500 s*uA
  MOSFETPriA2 : ee_lib/Semiconductors & Converters/Ideal Semiconductor Switch  port_option=ee.enum.controlport.ps  Ron=RdsOnPri_SI Ohm  Goff=GdsOffPri_SI 1/Ohm  Vth=VthPri_SI V  diode_param=ee.enum.semiconductors.protectionDiode.nodynamics  diode_Vf=VfPri_SI V  diode_Ron=RdPri_SI Ohm  diode_Goff=GdPri_SI 1/Ohm  diode_C=50e-9 F  diode_iRM=-235 A  diode_iF=300 A  diode_idot=-50 A/us  diode_trr_param=ee.enum.converters.diodetrr.trr_factor  diode_trr_factor=3  diode_trr=15 us  diode_Qrr=1500 s*uA
  MOSFETSecA1 : ee_lib/Semiconductors & Converters/Ideal Semiconductor Switch  port_option=ee.enum.controlport.ps  Ron=RdsOnSec_SI Ohm  Goff=GdsOffSec_SI 1/Ohm  Vth=VthSec_SI V  diode_param=ee.enum.semiconductors.protectionDiode.nodynamics  diode_Vf=VfSec_SI V  diode_Ron=RdSec_SI Ohm  diode_Goff=GdSec_SI 1/Ohm  diode_C=50e-9 F  diode_iRM=-235 A  diode_iF=300 A  diode_idot=-50 A/us  diode_trr_param=ee.enum.converters.diodetrr.trr_factor  diode_trr_factor=3  diode_trr=15 us  diode_Qrr=1500 s*uA
  MOSFETSecA2 : ee_lib/Semiconductors & Converters/Ideal Semiconductor Switch  port_option=ee.enum.controlport.ps  Ron=RdsOnSec_SI Ohm  Goff=GdsOffSec_SI 1/Ohm  Vth=VthSec_SI V  diode_param=ee.enum.semiconductors.protectionDiode.nodynamics  diode_Vf=VfSec_SI V  diode_Ron=RdSec_SI Ohm  diode_Goff=GdSec_SI 1/Ohm  diode_C=50e-9 F  diode_iRM=-235 A  diode_iF=300 A  diode_idot=-50 A/us  diode_trr_param=ee.enum.converters.diodetrr.trr_factor  diode_trr_factor=3  diode_trr=15 us  diode_Qrr=1500 s*uA
  MOSFETSecB1 : ee_lib/Semiconductors & Converters/Ideal Semiconductor Switch  port_option=ee.enum.controlport.ps  Ron=RdsOnSec_SI Ohm  Goff=GdsOffSec_SI 1/Ohm  Vth=VthSec_SI V  diode_param=ee.enum.semiconductors.protectionDiode.nodynamics  diode_Vf=VfSec_SI V  diode_Ron=RdSec_SI Ohm  diode_Goff=GdSec_SI 1/Ohm  diode_C=50e-9 F  diode_iRM=-235 A  diode_iF=300 A  diode_idot=-50 A/us  diode_trr_param=ee.enum.converters.diodetrr.trr_factor  diode_trr_factor=3  diode_trr=15 us  diode_Qrr=1500 s*uA
  MOSFETSecB2 : ee_lib/Semiconductors & Converters/Ideal Semiconductor Switch  port_option=ee.enum.controlport.ps  Ron=RdsOnSec_SI Ohm  Goff=GdsOffSec_SI 1/Ohm  Vth=VthSec_SI V  diode_param=ee.enum.semiconductors.protectionDiode.nodynamics  diode_Vf=VfSec_SI V  diode_Ron=RdSec_SI Ohm  diode_Goff=GdSec_SI 1/Ohm  diode_C=50e-9 F  diode_iRM=-235 A  diode_iF=300 A  diode_idot=-50 A/us  diode_trr_param=ee.enum.converters.diodetrr.trr_factor  diode_trr_factor=3  diode_trr=15 us  diode_Qrr=1500 s*uA
  Simulink-PS Converter{,1..7} (8 alike) : nesl_utility/Simulink-PS Converter  PhysicalDomain=network_engine_domain  SubClassName=ps_input  LeftPortType=input  RightPortType=output  PseudoPeriodic=off  Frequencies=[]  NoiseDistribution=none  NoiseParameters=[]  Unit=1  AffineConversion=off  FilteringAndDerivatives=provide  SimscapeFilterOrder=1  InputFilterTimeConstant=0.001  UdotUserProvided=0
  Transformer : ee_lib/Passive/Transformers/Mutual Inductor  L1=Lm_SI+Llk1_SI H  L2=Lm_SI/turnsRatio^2+Llk2_SI H  k=Lm_SI/sqrt((Lm_SI+Llk1_SI)*(Lm_SI+turnsRatio^2*Llk2_SI))  L_tol=0  enable_L1_tol=ee.enum.toleranceApplication.none  L1_tol_distribution=ee.enum.toleranceDistribution.uniform  L1_nSigma=4  enable_L2_tol=ee.enum.toleranceApplication.none  L2_tol_distribution=ee.enum.toleranceDistribution.uniform  L2_nSigma=4  r=[RLlk1_SI, RLlk2_SI] Ohm  g=[1e-09, 1e-09] 1/Ohm  enable_operating_limits=ee.enum.enable.no  operating_limit_action=ee.enum.passive.reportOpLim.warn  max_working_current=1 A  power_rating=1 W  iL1_specify=off  iL1_priority=High  iL1=0 A  iL1_nominal_specify=off  iL1_nominal_value=1  iL1_nominal_unit=A  iL2_specify=off  iL2_priority=High  iL2=0 A  iL2_nominal_specify=off  iL2_nominal_value=1  iL2_nominal_unit=A
  VinSens : Subsystem
      mask Display: disp('V')
  VoutSens : Subsystem
      settings: PortSchema="{\"entries\":[{\"content\":{\"sides\":[{\"content\":{\"connectorIds\":[\"LConn1\"]},\"type\":\"ConnectorPlacement.EquallySpacedRectSide\",\"uuid\":\"da66b42d-39ba-4e5d-9b19-dc680792542d\"},{\"content\":{\"connectorIds\":[\"RConn1\",\"Out1\"],\"side\":\"RIGHT\"},\"type\":\"ConnectorPlacement.EquallySpacedRectSide\",\"uuid\":\"9a34d54a-b1f0-405a-82c9-4333c7864e33\"},{\"content\":{\"side\":\"TOP\"},\"type\":\"ConnectorPlacement.EquallySpacedRectSide\",\"uuid\":\"3d98f795-d173-4072-aa84-47617691d0d7\"}]},\"type\":\"ConnectorPlacement.EquallySpacedConnector\",\"uuid\":\"cc1a3107-18f6-4c4b-a82f-56637250e4a4\"}],\"packageUris\":[\"http://schema.mathworks.com/mf0/Connector/R2020b\"],\"version\":\"1.0\"}"
      mask Display: disp('V')
  Vin+ : PMIOPort  Side=Left
  Vin- : PMIOPort  Port=2  Side=Left
  Vout+ : PMIOPort  Port=3  Side=Right
  Vout- : PMIOPort  Port=4  Side=Right
  Out Bus Element1 : Outport  PortName=meas  Element=Ip [A]
  Out Bus Element2 : Outport  PortName=meas  Element=Is [A]
  Out Bus Element3 : Outport  PortName=meas  Element=Vin [V]
  Out Bus Element4 : Outport  PortName=meas  Element=Vout [V]
  Out Bus Element5 : Outport  PortName=meas  Element=Iin [A]
  Out Bus Element6 : Outport  PortName=meas  Element=Iout [A]
  wires:
  Gp/1 -> Demux/1
  Demux/1 -> [G1]
  Demux/2 -> [G2]
  Demux/3 -> [G3]
  Demux/4 -> [G4]
  Demux1/1 -> [G5]
  Demux1/2 -> [G6]
  Demux1/3 -> [G7]
  Demux1/4 -> [G8]
  [G2] -> Simulink-PS Converter1/1
  Iin/1(I) -> Out Bus Element5/1
  Iout/1(I) -> Out Bus Element6/1
  Ip/1(I) -> Out Bus Element1/1
  Is/1(I) -> Out Bus Element2/1
  VinSens/1(V) -> Out Bus Element3/1
  VoutSens/1(V) -> Out Bus Element4/1
  [G1] -> Simulink-PS Converter/1
  [G3] -> Simulink-PS Converter2/1
  [G4] -> Simulink-PS Converter3/1
  [G5] -> Simulink-PS Converter4/1
  [G6] -> Simulink-PS Converter5/1
  [G7] -> Simulink-PS Converter6/1
  [G8] -> Simulink-PS Converter7/1
  Gs/1 -> Demux1/1
  connections:
  MOSFETPriA1/RConn2 -- Ip/LConn1 -- MOSFETPriA2/RConn1
  Simulink-PS Converter/RConn1 -- MOSFETPriA1/LConn1
  Simulink-PS Converter1/RConn1 -- MOSFETPriA2/LConn1
  Simulink-PS Converter2/RConn1 -- MOSFETB1/LConn1
  Simulink-PS Converter3/RConn1 -- MOSFETB2/LConn1
  MOSFETB1/RConn2 -- Transformer/LConn2 -- MOSFETB2/RConn1
  Vin+/RConn1 -- Iin/LConn1 -- VinSens/LConn1
  VinSens/RConn1 -- Vin-/RConn1 -- MOSFETB2/RConn2 -- MOSFETPriA2/RConn2
  MOSFETSecA1/RConn2 -- Is/RConn1 -- MOSFETSecA2/RConn1
  Ip/RConn1 -- Lr/LConn1
  Transformer/LConn1 -- Lr/RConn1
  Is/LConn1 -- Transformer/RConn1
  Simulink-PS Converter4/RConn1 -- MOSFETSecA1/LConn1
  Simulink-PS Converter5/RConn1 -- MOSFETSecA2/LConn1
  MOSFETSecA1/RConn1 -- Iout/LConn1 -- Co/LConn1 -- MOSFETSecB1/RConn1
  MOSFETSecB1/RConn2 -- Transformer/RConn2 -- MOSFETSecB2/RConn1
  Simulink-PS Converter6/RConn1 -- MOSFETSecB1/LConn1
  Simulink-PS Converter7/RConn1 -- MOSFETSecB2/LConn1
  MOSFETSecB2/RConn2 -- VoutSens/RConn1 -- Vout-/RConn1 -- Co/RConn1 -- MOSFETSecA2/RConn2
  Iout/RConn1 -- Vout+/RConn1 -- VoutSens/LConn1
  MOSFETPriA1/RConn1 -- MOSFETB1/RConn1 -- Iin/RConn1

== system DABTestHarnessPlant/DAB PWM Generator/Ramp Mode/FixedStep ==
  Tsw : Inport
  Initial Ramp Value : InitialCondition  Value=0
  Overshoot Residual : Sum  Inputs=-+
  Period Reached : RelationalOperator  Operator=>  ZeroCross=off
  Time Ramp : DiscreteIntegrator  ExternalReset=rising  InitialConditionSource=external  SampleTime=Ts  ShowStatePort=on  ICPrevOutput=DiscIntNeverNeededParam  ICPrevScaledInput=DiscIntNeverNeededParam
  Unit Rate : Constant
  S : Outport
  wires:
  Initial Ramp Value/1 -> Time Ramp/3
  Overshoot Residual/1 -> Initial Ramp Value/1
  Time Ramp/State -> Overshoot Residual/2, Period Reached/1
  Tsw/1 -> Period Reached/2, Overshoot Residual/1
  Time Ramp/1 -> S/1
  Period Reached/1 -> Time Ramp/2
  Unit Rate/1 -> Time Ramp/1

== system DABTestHarnessPlant/DAB PWM Generator/Ramp Mode/VariableStep ==
  Tsw : Inport
  Initial Ramp Value : InitialCondition  Value=0
  Overshoot Residual : Sum  Inputs=-+
  Period Reached : RelationalOperator  Operator=>
  Time Ramp : Integrator  ExternalReset=rising  InitialConditionSource=external  ShowStatePort=on
  Unit Rate : Constant
  S : Outport
  wires:
  Initial Ramp Value/1 -> Time Ramp/3
  Overshoot Residual/1 -> Initial Ramp Value/1
  Time Ramp/State -> Overshoot Residual/2, Period Reached/1
  Tsw/1 -> Period Reached/2, Overshoot Residual/1
  Time Ramp/1 -> S/1
  Period Reached/1 -> Time Ramp/2
  Unit Rate/1 -> Time Ramp/1

== system DABTestHarnessPlant/DAB Converter/DABConverterVariant/DetailedModel/Iin ==
  Current Sensor : fl_lib/Electrical/Electrical Sensors/Current Sensor
  PS-Simulink Converter : nesl_utility/PS-Simulink Converter  PhysicalDomain=network_engine_domain  SubClassName=ps_output  LeftPortType=input  RightPortType=output  PseudoPeriodic=off  Frequencies=[]  VectorFormat=inherit  Unit=inherit  AffineConversion=off
  + : PMIOPort  Side=Left
  - : PMIOPort  Port=2  Side=Right
  I : Outport
  wires:
  PS-Simulink Converter/1 -> I/1
  connections:
  Current Sensor/RConn1 -- PS-Simulink Converter/LConn1
  Current Sensor/RConn2 -- -/RConn1
  +/RConn1 -- Current Sensor/LConn1

== system DABTestHarnessPlant/DAB Converter/DABConverterVariant/DetailedModel/Iout ==
  Current Sensor : fl_lib/Electrical/Electrical Sensors/Current Sensor
  PS-Simulink Converter : nesl_utility/PS-Simulink Converter  PhysicalDomain=network_engine_domain  SubClassName=ps_output  LeftPortType=input  RightPortType=output  PseudoPeriodic=off  Frequencies=[]  VectorFormat=inherit  Unit=inherit  AffineConversion=off
  + : PMIOPort  Side=Left
  - : PMIOPort  Port=2  Side=Right
  I : Outport
  wires:
  PS-Simulink Converter/1 -> I/1
  connections:
  Current Sensor/RConn1 -- PS-Simulink Converter/LConn1
  Current Sensor/RConn2 -- -/RConn1
  +/RConn1 -- Current Sensor/LConn1

== system DABTestHarnessPlant/DAB Converter/DABConverterVariant/DetailedModel/Ip ==
  Current Sensor : fl_lib/Electrical/Electrical Sensors/Current Sensor
  PS-Simulink Converter : nesl_utility/PS-Simulink Converter  PhysicalDomain=network_engine_domain  SubClassName=ps_output  LeftPortType=input  RightPortType=output  PseudoPeriodic=off  Frequencies=[]  VectorFormat=inherit  Unit=inherit  AffineConversion=off
  + : PMIOPort  Side=Left
  - : PMIOPort  Port=2  Side=Right
  I : Outport
  wires:
  PS-Simulink Converter/1 -> I/1
  connections:
  Current Sensor/RConn1 -- PS-Simulink Converter/LConn1
  Current Sensor/RConn2 -- -/RConn1
  +/RConn1 -- Current Sensor/LConn1
